simulink model "furuta_single_inverted_pendulum_model_CL_PD_Initial"  (R2025a)
settings: Solver=ode4  StartTime=0.0  StopTime=inf  FixedStep=Ts  RelTol=1e-3
InitFcn:
  | addpath('functions');
model workspace (MATLAB code in the model file):
  | arm_torque = 0;
  | L_arm = 0.2;
  | I_arm = 0.01;
  | lcom_1 = 0.6;
  | I_1 = 0.02;
  | m_1 = 1;
  | L_1 = 1;
  | 
  | init_cond = [pi/2; 0; 0.01; 0];
undefined symbols (not defined in the file or in its folder): DiscIntNeverNeededParam, Kd_ArmAngle, Kd_ArmVelocity, Kd_PendulumAngle, Kd_PendulumVelocity, Ts
settings Model: Creator=Esther  LastModifiedBy=marcus

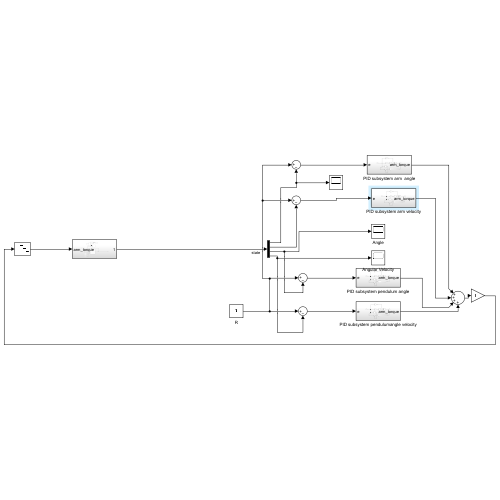
[thumbnail: Simulink's stored preview of the top-level diagram]
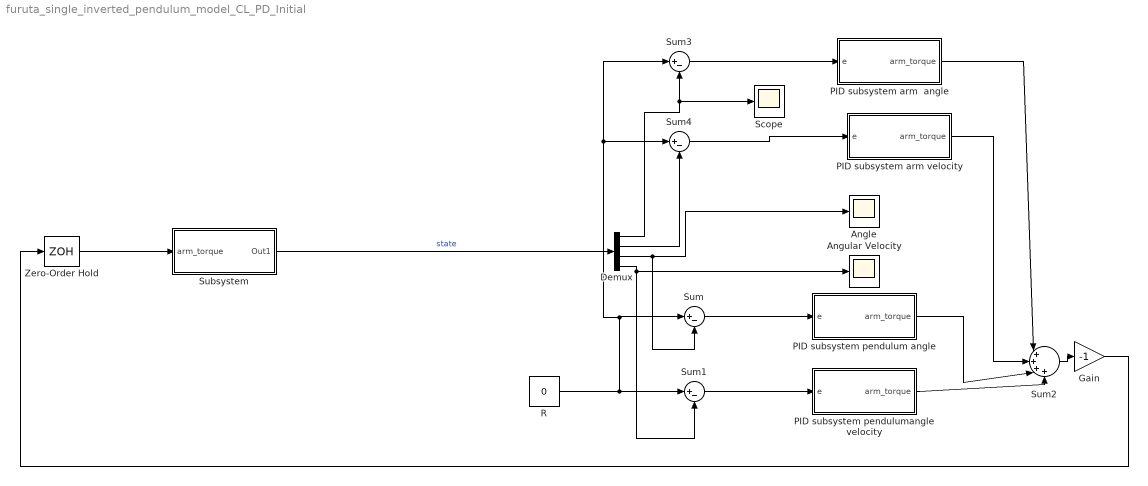
== system furuta_single_inverted_pendulum_model_CL_PD_Initial ==
  Angle : Scope
      settings: ActiveDisplayYMinimum=-6.9679733150236753  ActiveDisplayYMaximum=4.0512303756780108
  Angular Velocity : Scope
      settings: ActiveDisplayYMinimum=-3875.8658390527003  ActiveDisplayYMaximum=3642.7464695660938  DataLoggingVariableName=ScopeData2
  Demux : Demux
  Gain : Gain  Gain=-1
  PID subsystem arm  angle : Subsystem
  PID subsystem arm velocity : Subsystem
  PID subsystem pendulum angle : Subsystem
  PID subsystem pendulumangle velocity : Subsystem
  R : Constant  Value=0
  Scope : Scope
      settings: ActiveDisplayYMinimum=0.66987931121046485  ActiveDisplayYMaximum=9.6235763800171945
  Subsystem : Subsystem
  Sum{,1,3..4} (4 alike) : Sum  Inputs=|+-
  Sum2 : Sum  Inputs=|++++
  Zero-Order Hold : ZeroOrderHold  SampleTime=Ts
  wires:
  Subsystem/1(Out1) -> Demux/1  "state"
  R/1 -> Sum1/1, Sum3/1, Sum4/1, Sum/1
  Demux/3 -> Angle/1, Sum/2
  Demux/4 -> Angular Velocity/1, Sum1/2
  Sum2/1 -> Gain/1
  PID subsystem arm  angle/1(arm_torque) -> Sum2/1
  Demux/1 -> Scope/1, Sum3/2
  Demux/2 -> Sum4/2
  Gain/1 -> Zero-Order Hold/1
  Zero-Order Hold/1 -> Subsystem/1(arm_torque)
  Sum1/1 -> PID subsystem pendulumangle velocity/1(e)
  PID subsystem pendulumangle velocity/1(arm_torque) -> Sum2/4
  Sum/1 -> PID subsystem pendulum angle/1(e)
  PID subsystem pendulum angle/1(arm_torque) -> Sum2/3
  Sum4/1 -> PID subsystem arm velocity/1(e)
  Sum3/1 -> PID subsystem arm  angle/1(e)
  PID subsystem arm velocity/1(arm_torque) -> Sum2/2

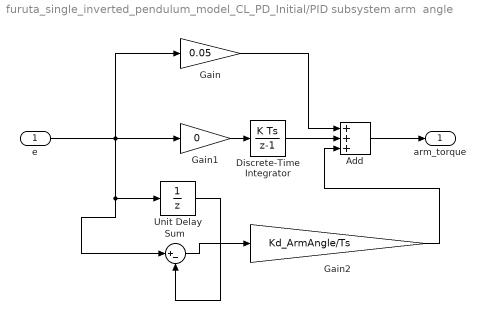
== system furuta_single_inverted_pendulum_model_CL_PD_Initial/PID subsystem arm  angle ==
  e : Inport
  Add : Sum  Inputs=+++
  Discrete-Time Integrator : DiscreteIntegrator  gainval=1  SampleTime=0.001  ICPrevOutput=DiscIntNeverNeededParam  ICPrevScaledInput=DiscIntNeverNeededParam
  Gain : Gain  Gain=0.05
  Gain1 : Gain  Gain=0
  Gain2 : Gain  Gain=Kd_ArmAngle/Ts
  Sum : Sum  Inputs=|+-
  Unit Delay : UnitDelay  SampleTime=-1  HasFrameUpgradeWarning=on
  arm_torque : Outport
  wires:
  e/1 -> Sum/1, Unit Delay/1, Gain/1, Gain1/1
  Unit Delay/1 -> Sum/2
  Discrete-Time Integrator/1 -> Add/2
  Gain/1 -> Add/1
  Add/1 -> arm_torque/1
  Gain1/1 -> Discrete-Time Integrator/1
  Gain2/1 -> Add/3
  Sum/1 -> Gain2/1

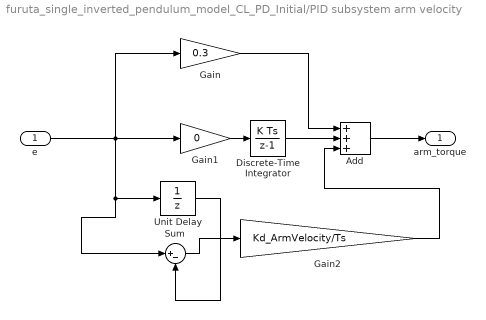
== system furuta_single_inverted_pendulum_model_CL_PD_Initial/PID subsystem arm velocity ==
  e : Inport
  Add : Sum  Inputs=+++
  Discrete-Time Integrator : DiscreteIntegrator  gainval=1  SampleTime=0.001  ICPrevOutput=DiscIntNeverNeededParam  ICPrevScaledInput=DiscIntNeverNeededParam
  Gain : Gain  Gain=0.3
  Gain1 : Gain  Gain=0
  Gain2 : Gain  Gain=Kd_ArmVelocity/Ts
  Sum : Sum  Inputs=|+-
  Unit Delay : UnitDelay  SampleTime=-1  HasFrameUpgradeWarning=on
  arm_torque : Outport
  wires:
  e/1 -> Sum/1, Unit Delay/1, Gain/1, Gain1/1
  Unit Delay/1 -> Sum/2
  Discrete-Time Integrator/1 -> Add/2
  Gain/1 -> Add/1
  Add/1 -> arm_torque/1
  Gain1/1 -> Discrete-Time Integrator/1
  Gain2/1 -> Add/3
  Sum/1 -> Gain2/1

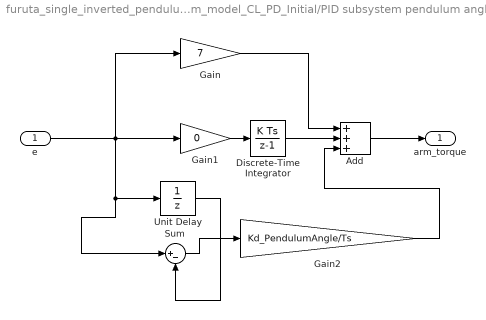
== system furuta_single_inverted_pendulum_model_CL_PD_Initial/PID subsystem pendulum angle ==
  e : Inport
  Add : Sum  Inputs=+++
  Discrete-Time Integrator : DiscreteIntegrator  gainval=1  SampleTime=0.001  ICPrevOutput=DiscIntNeverNeededParam  ICPrevScaledInput=DiscIntNeverNeededParam
  Gain : Gain  Gain=7
  Gain1 : Gain  Gain=0
  Gain2 : Gain  Gain=Kd_PendulumAngle/Ts
  Sum : Sum  Inputs=|+-
  Unit Delay : UnitDelay  SampleTime=-1  HasFrameUpgradeWarning=on
  arm_torque : Outport
  wires:
  e/1 -> Sum/1, Unit Delay/1, Gain/1, Gain1/1
  Unit Delay/1 -> Sum/2
  Discrete-Time Integrator/1 -> Add/2
  Gain/1 -> Add/1
  Add/1 -> arm_torque/1
  Gain1/1 -> Discrete-Time Integrator/1
  Gain2/1 -> Add/3
  Sum/1 -> Gain2/1

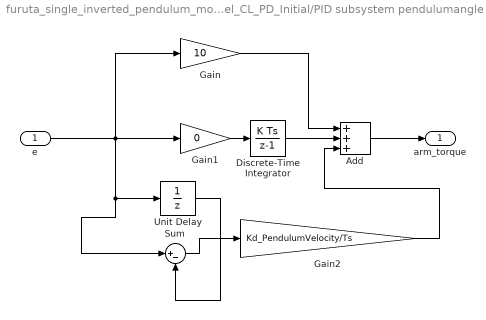
== system furuta_single_inverted_pendulum_model_CL_PD_Initial/PID subsystem pendulumangle velocity ==
  e : Inport
  Add : Sum  Inputs=+++
  Discrete-Time Integrator : DiscreteIntegrator  gainval=1  SampleTime=0.001  ICPrevOutput=DiscIntNeverNeededParam  ICPrevScaledInput=DiscIntNeverNeededParam
  Gain : Gain  Gain=10
  Gain1 : Gain  Gain=0
  Gain2 : Gain  Gain=Kd_PendulumVelocity/Ts
  Sum : Sum  Inputs=|+-
  Unit Delay : UnitDelay  SampleTime=-1  HasFrameUpgradeWarning=on
  arm_torque : Outport
  wires:
  e/1 -> Sum/1, Unit Delay/1, Gain/1, Gain1/1
  Unit Delay/1 -> Sum/2
  Discrete-Time Integrator/1 -> Add/2
  Gain/1 -> Add/1
  Add/1 -> arm_torque/1
  Gain1/1 -> Discrete-Time Integrator/1
  Gain2/1 -> Add/3
  Sum/1 -> Gain2/1

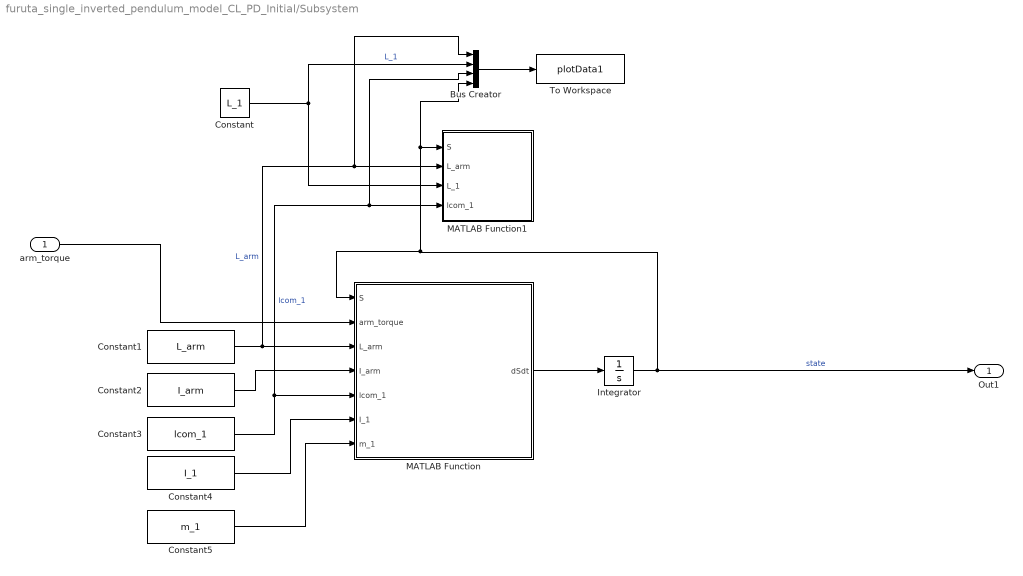
== system furuta_single_inverted_pendulum_model_CL_PD_Initial/Subsystem ==
  arm_torque : Inport
  Bus Creator : BusCreator  Inputs=4
  Constant : Constant  Value=L_1
  Constant1 : Constant  Value=L_arm
  Constant2 : Constant  Value=I_arm
  Constant3 : Constant  Value=lcom_1
  Constant4 : Constant  Value=I_1
  Constant5 : Constant  Value=m_1
  Integrator : Integrator  InitialCondition=init_cond
  MATLAB Function : MATLAB Function  TreatAsAtomicUnit=on
  MATLAB Function1 : MATLAB Function  TreatAsAtomicUnit=on
  To Workspace : ToWorkspace  VariableName=plotData1  SaveFormat=Timeseries  SampleTime=-1
  Out1 : Outport
  wires:
  Bus Creator/1 -> To Workspace/1
  Constant/1 -> Bus Creator/2, MATLAB Function1/3(L_1)  "L_1"
  Constant2/1 -> MATLAB Function/4(I_arm)
  Constant4/1 -> MATLAB Function/6(I_1)
  Constant1/1 -> MATLAB Function/3(L_arm), Bus Creator/1, MATLAB Function1/2(L_arm)  "L_arm"
  Integrator/1 -> Out1/1, MATLAB Function/1(S), MATLAB Function1/1(S), Bus Creator/4  "state"
  Constant3/1 -> Bus Creator/3, MATLAB Function1/4(lcom_1), MATLAB Function/5(lcom_1)  "lcom_1"
  Constant5/1 -> MATLAB Function/7(m_1)
  arm_torque/1 -> MATLAB Function/2(arm_torque)
  MATLAB Function/1(dSdt) -> Integrator/1

== matlab function furuta_single_inverted_pendulum_model_CL_PD_Initial/Subsystem/MATLAB Function ==
  data: S input size=4; dSdt output size=4; arm_torque input size=1; L_arm input size=1; I_arm input size=1; lcom_1 input size=1; I_1 input size=1; m_1 input size=1
function dSdt = get_dSdt(S, arm_torque, L_arm, I_arm, lcom_1, I_1, m_1)
    t = 0;
    g = 9.81;
    phys_param = [L_arm, I_arm, lcom_1, I_1, m_1, g];
    fric_arm = [0.018, 0.018, 100];
    fric_1 = [0.0001, 0.0001, 100];
    dSdt = furuta_single_state_derivative(t, S, arm_torque, phys_param, fric_arm, fric_1);
end

== matlab function furuta_single_inverted_pendulum_model_CL_PD_Initial/Subsystem/MATLAB Function1 ==
  settings: updateMethod=DISCRETE
  data: S input; L_arm input; L_1 input; lcom_1 input
function animation(S, L_arm, L_1, lcom_1)
    update_ratio = 100;
    realtime_animation_single(S, L_arm, L_1, lcom_1, update_ratio);
end
